simulink model "PV100_wattsANN"  (R2016a)
settings: Solver=ode45  StartTime=0.0  StopTime=0.5  RelTol=1e-3
undefined symbols (not defined in the file or in its folder): anpv1
libraries: powerlib x10, fuzblock x1, re_lib x1, powerlib_extras x1
settings Model: Creator=Indhu  LastModifiedBy=yaju
settings DataIOCC: LimitDataPoints=on  SaveFormat=Array  InspectSignalLogs=on
settings DebuggingCC: SolverPrmCheckMsg=warning
settings HardwareCC: ProdBitPerPointer=32  ProdLargestAtomicFloat=None  ProdIntDivRoundTo=Undefined  ProdEndianess=Unspecified  ProdWordSize=32  ProdHWDeviceType=32-bit Generic
settings ModelReferenceCC: PropagateSignalLabelsOutOfModel=off
settings ConfigComp: CovModelRefEnable=Off  CovSFcnEnable=off

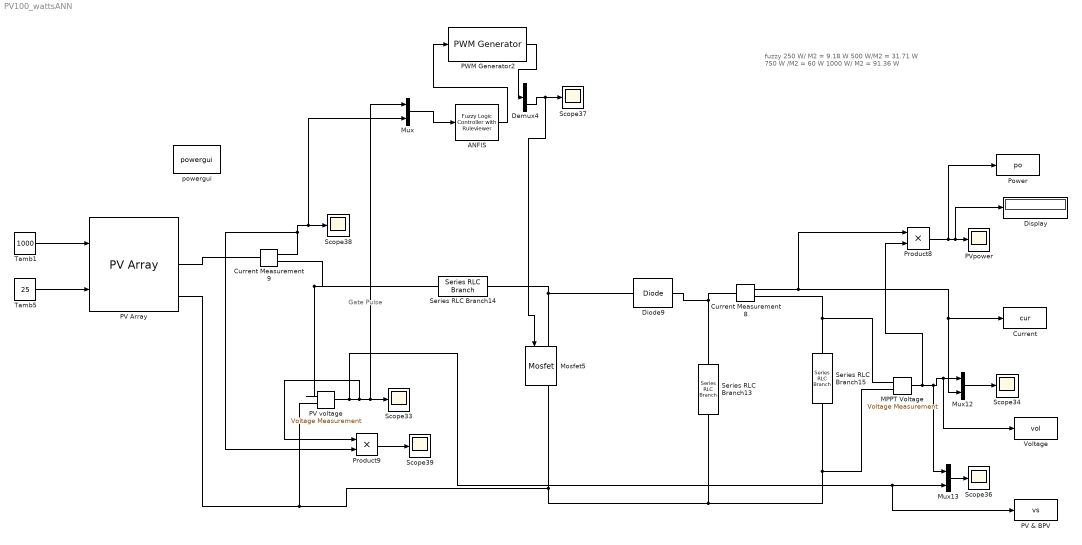
== system PV100_wattsANN ==
  note: fuzzy
      | 250 W/ M2 = 9.18 W
      | 500 W/M2 = 31.71 W
      | 750 W /M2 = 60 W
      | 1000 W/ M2 = 91.36 W
  note: Gate Pulse
  ANFIS : fuzblock/Fuzzy Logic  Controller  with Ruleviewer  fismatrix=[anpv1]  Ts=0.001
  Current : ToWorkspace  VariableName=cur  SaveFormat=Timeseries  SampleTime=-1
  Current Measurement8 : powerlib/Measurements/Current Measurement  PhasorSimulation=off  OutputType=Complex  PSBequivalent=0
  Current Measurement9 : powerlib/Measurements/Current Measurement  PhasorSimulation=off  OutputType=Complex  PSBequivalent=0
  Demux4 : Demux  Outputs=2
  Diode9 : powerlib/Power Electronics/Diode  Ron=0.001  Lon=0  Vf=0.8  IC=0  UseSnubber=off  Rs=500  Cs=250e-9  Measurements=off
  Display : Display
  "MPPT Voltage " : powerlib/Measurements/Voltage Measurement  PhasorSimulation=off  OutputType=Complex  PSBequivalent=0
  Mosfet5 : powerlib/Power Electronics/Mosfet  Ron=0.1  Lon=0  Rd=0.01  Vfd=0  IC=0  Rs=1e5  Cs=inf  Measurements=on
  Mux : Mux  Inputs=2
  Mux12 : Mux  Inputs=2
  Mux13 : Mux  Inputs=2
  PV & BPV : ToWorkspace  VariableName=vs  SaveFormat=Timeseries  SampleTime=-1
  PV Array : re_lib/Solar/PV Array  Npar=1  Nser=1  PlotType=array @ 25 deg.C & specified irradiances  S_vec="[ 1000  750  500  250 ]"  Temp_C_vec=[25]  ModuleName=User-defined  PlotWhenSelected=off  Pm=100.45  Ncell=60  Voc=22  Isc=5.2  Vm=20.5  Im=4.9  beta_Voc_pc=-0.369  alpha_Isc_pc=0.091995  beta_Voc=-0.08118  alpha_Isc=0.0047837  IL=5.2001  I0=5.4941e-07  nI=1.0022  Rsh=136.667  Rs=0.040204  BAL=off  Tc=1e-6  Tfilter=5e-5
  "PV voltage " : powerlib/Measurements/Voltage Measurement  PhasorSimulation=off  OutputType=Complex  PSBequivalent=0
  PVpower : Scope
  PWM Generator2 : powerlib_extras/Control  Blocks/PWM Generator  GeneratorMode="1-arm  bridge (2 pulses)"  Fc=3000  Internal=off  mIndex=0.4  Freq=50  Phase=0
  Power : ToWorkspace  VariableName=po  SaveFormat=Timeseries  SampleTime=-1
  Product8 : Product  RndMeth=Zero
  Product9 : Product  RndMeth=Zero
  Scope{33..34,36..39} (6 alike) : Scope
  Series RLC Branch13 : powerlib/Elements/Series RLC Branch  LConnTagsString=__new0  RConnTagsString=__new0  BranchType=C  Resistance=1  Inductance=1e-3  SetiL0=off  InitialCurrent=0  Capacitance=550e-6  Setx0=off  InitialVoltage=0  Measurements=None
  Series RLC Branch14 : powerlib/Elements/Series RLC Branch  LConnTagsString=__new0  RConnTagsString=__new0  BranchType=L  Resistance=1  Inductance=161e-3  SetiL0=off  InitialCurrent=0  Capacitance=1e-6  Setx0=off  InitialVoltage=0  Measurements=None
  Series RLC Branch15 : powerlib/Elements/Series RLC Branch  LConnTagsString=__new0  RConnTagsString=__new0  BranchType=R  Resistance=6.5  Inductance=1e-3  SetiL0=off  InitialCurrent=0  Capacitance=1e-6  Setx0=off  InitialVoltage=0  Measurements=None
  Tamb1 : Constant  Value=1000
  Tamb5 : Constant  Value=25
  Voltage : ToWorkspace  VariableName=vol  SaveFormat=Timeseries  SampleTime=-1
  powergui : powerlib/powergui  Priority=1  SimulationMode=Discrete  SolverType=Tustin  SampleTime=1e-6  frequency=60  SPID=off  DisableSnubberDevices=off  DisableRonSwitches=off  DisableVfSwitches=off  SwTol=0  DisplayEquations=off  Interpol=off  ExternalGateDelay=off  methode=off  Ts=0  FunctionMessages=off  echomessages=off  HookPort=off  EnableUseOfTLC=off  x0status=blocks  frequencyindice=0  Pbase=100e6  ErrMax=1e-4  Iterations=50  UnitsV=kV  UnitsW=MW  buscounter=0  RestoreLinks=warning  ResistiveCurrentMeasurement=off  Frange=[0:2:500]  Ylog=off  Xlog=on  ShowGrid=off  save=off  variable=ZData  structure=0  ZoomFFT=off  StartTime=0.0  cycles=1  DisplayStyle=1  fundamental=60  FreqAxis=off  MaxFrequency=1000  frequencyindicesteady=1  RmsSteady=1  display=off
  wires:
  PWM Generator2/1 -> Demux4/1
  Current Measurement8/1 -> Current/1, Mux12/2, Product8/1
  "MPPT Voltage "/1 -> Voltage/1, Mux12/1, Mux13/1, Product8/2
  Mux12/1 -> Scope34/1
  Mux13/1 -> Scope36/1
  Product8/1 -> Display/1, PVpower/1, Power/1
  Product9/1 -> Scope39/1
  Tamb5/1 -> PV Array/2
  Tamb1/1 -> PV Array/1
  "PV voltage "/1 -> PV & BPV/1, Mux13/2, Product9/1, Mux/1, Scope33/1
  Current Measurement9/1 -> Product9/2, Mux/2, Scope38/1
  ANFIS/1 -> PWM Generator2/1
  Mux/1 -> ANFIS/1
  Demux4/2 -> Mosfet5/1, Scope37/1
  connections:
  Series RLC Branch14/RConn1 -- Mosfet5/LConn1 -- Diode9/LConn1
  Diode9/RConn1 -- Current Measurement8/LConn1 -- Series RLC Branch13/LConn1
  Current Measurement8/RConn1 -- "MPPT Voltage "/LConn1 -- Series RLC Branch15/LConn1
  "PV voltage "/LConn1 -- Series RLC Branch14/LConn1 -- Current Measurement9/RConn1
  Mosfet5/RConn1 -- Series RLC Branch15/RConn1 -- "MPPT Voltage "/LConn2 -- Series RLC Branch13/RConn1 -- PV Array/RConn2 -- "PV voltage "/LConn2
  Current Measurement9/LConn1 -- PV Array/RConn1
